simulink model "Full_System"  (R2024a)
settings: Solver=FixedStepDiscrete  StartTime=0.0  StopTime=10.0  RelTol=1e-3
undefined symbols (not defined in the file): Ion, Lithium
libraries: spsSeriesRLCBranchLib x6, spsBuckConverterLib x2, spsCurrentMeasurementLib x2, spsBatteryLib x1, spsPWMGeneratorDCDCLib x1, spsGroundLib x1, spsPVArrayLib x1, eePwmGenerator x1, spsVoltageMeasurementLib x1, spspowerguiLib x1
settings Model: Creator=KennyBoum-biha  LastModifiedBy=k_boumbi
settings DebuggingCC: UnconnectedInputMsg=warning  UnconnectedOutputMsg=warning  UnconnectedLineMsg=warning
settings ModelReferenceCC: EnableRefExpFcnMdlSchedulingChecks=on
settings RTWCC: GPUComputeCapability=3.5  DLArmComputeVersion=19.05

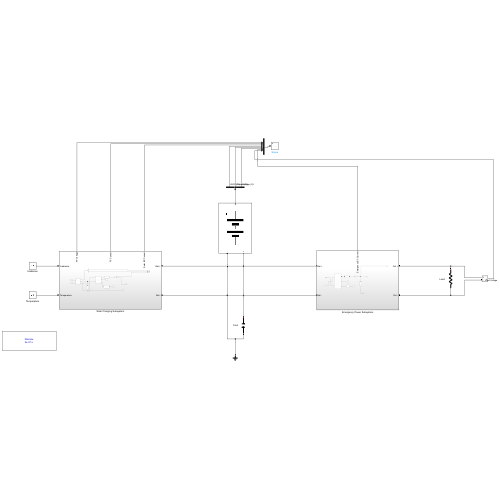
[thumbnail: Simulink's stored preview of the top-level diagram]
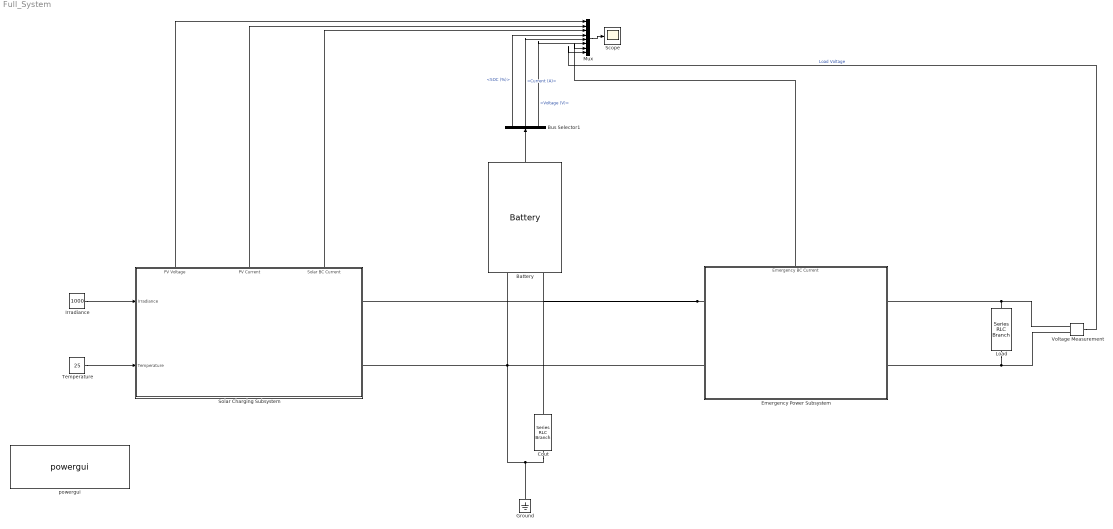
== system Full_System ==
  Battery : spsBatteryLib/Battery  BatType=Lithium-Ion  ShowTempParam=off  ThermalPreset=no  ShowAgeParam=off  NomV=48  NomQ=0.5  SOC=50  Batt_Tr=5  PresetModel=on  MaxQ=0.5  MinV=36  FullV=55.8714  Dis_rate=0.21739  R=0.96  Normal_OP=0.45217  expZone="[51.8585    0.0245652]"  current=[6.5 13 32.5]  Units=Time  Tci=20  NomT=20  T2=-30  MaxQ2=4.8  FullV2=7.1  Normal_OP2=5.655  expZone2="[6.58           1]"  Rca=0.6  ti=2000  Dp=0  Neq0=0  Tsim=1e6  Ta1=25  Qeol=5.4*0.9  Reol=0.013333*1.2  Char_age=[2.3478, 3]  Dis_age=[2.3478, 10]  N1=1500  N2=10500  N3=1000  N4=1400  Ta2=45  N5=950
  Bus Selector1 : BusSelector  OutputSignals=SOC (%),Current (A),Voltage (V)
  Cout : spsSeriesRLCBranchLib/Series RLC Branch  LConnTagsString=__new0  RConnTagsString=__new0  BranchType=C  Resistance=1  Inductance=47e-6  SetiL0=off  InitialCurrent=0  Capacitance=100e-6  Setx0=off  InitialVoltage=0  Measurements=None
  Emergency Power Subsystem : Subsystem
      settings: PortSchema="{\"entries\":[{\"content\":{\"sides\":[{\"content\":{\"connectorIds\":[\"LConn1\",\"LConn2\"]},\"type\":\"ConnectorPlacement.EquallySpacedRectSide\",\"uuid\":\"cf3750f3-3e81-4659-820f-f75c62c5389c\"},{\"content\":{\"connectorIds\":[\"RConn1\",\"RConn2\"],\"side\":\"RIGHT\"},\"type\":\"ConnectorPlacement.EquallySpacedRectSide\",\"uuid\":\"3e630a51-3c98-4ea6-b09a-757b6c47ec4c\"},{\"content\":{\"connectorIds\":[\"Out1\"],\"side\":\"TOP\"},\"type\":\"ConnectorPlacement.EquallySpacedRectSide\",\"uuid\":\"d6b0d433-2319-4baf-b8a3-4fb876102fd6\"}]},\"type\":\"ConnectorPlacement.EquallySpacedConnector\",\"uuid\":\"13c5517f-e21d-46a3-ac40-d14bb8a08b57\"}],\"packageUris\":[\"http://schema.mathworks.com/mf0/Connector/R2020b\"],\"version\":\"1.0\"}"
  Ground : spsGroundLib/Ground  LConnTagsString=a
  Irradiance : Constant  Value=1000
  Load : spsSeriesRLCBranchLib/Series RLC Branch  LConnTagsString=__new0  RConnTagsString=__new0  BranchType=R  Resistance=1.44  Inductance=1e-3  SetiL0=off  InitialCurrent=0  Capacitance=1e-6  Setx0=off  InitialVoltage=0  Measurements=None
  Mux : Mux  Inputs=8
  Scope : Scope
  Solar Charging Subsystem : Subsystem
      settings: PortSchema="{\"entries\":[{\"content\":{\"sides\":[{\"content\":{\"connectorIds\":[\"In1\",\"In2\"]},\"type\":\"ConnectorPlacement.EquallySpacedRectSide\",\"uuid\":\"cb229151-0742-4502-9ccd-990ff05f6a8c\"},{\"content\":{\"connectorIds\":[\"RConn1\",\"RConn2\"],\"side\":\"RIGHT\"},\"type\":\"ConnectorPlacement.EquallySpacedRectSide\",\"uuid\":\"9e14cc4e-58f0-4588-8f9d-a6a650a5df1b\"},{\"content\":{\"connectorIds\":[\"Out1\",\"Out2\",\"Out3\"],\"side\":\"TOP\"},\"type\":\"ConnectorPlacement.EquallySpacedRectSide\",\"uuid\":\"ec81657c-9ee6-4126-bdd0-5a56d1ba93e0\"}]},\"type\":\"ConnectorPlacement.EquallySpacedConnector\",\"uuid\":\"153089d4-0393-4364-aaa8-7b9cfec9044a\"}],\"packageUris\":[\"http://schema.mathworks.com/mf0/Connector/R2020b\"],\"version\":\"1.0\"}"
  Temperature : Constant  Value=25
  Voltage Measurement : spsVoltageMeasurementLib/Voltage Measurement  PhasorSimulation=off  OutputType=Complex  PSBequivalent=0
  powergui : spspowerguiLib/powergui  Priority=1  SimulationMode=Discrete  SampleTime=2e-7  frequency=60  Iterations=50  frequencyindice=0  Pbase=100e6  ErrMax=1e-4  UnitsV=kV  UnitsW=MW  buscounter=0  FunctionMessages=off  echomessages=off  EnableUseOfTLC=off  CurrentSourceSwitches=off  DisableSnubberDevices=off  DisableRonSwitches=off  DisableVfSwitches=off  DisplayEquations=off  AutomaticDiscreteSolvers=off  SolverType=Tustin/Backward Euler (TBE)  Interpol=off  ExternalGateDelay=off  methode=off  Ts=100  x0status=blocks  SPID=on  SwTol=0  HookPort=off  NonlinearTolerance=1e-4  nMaxIteration=100  ContinueOnMaxIteration=off  RestoreLinks=warning  ResistiveCurrentMeasurement=off  Frange=[0:2:500]  Ylog=off  Xlog=on  ShowGrid=off  save=off  variable=ZData  structure=0  ZoomFFT=off  StartTime=0.0  cycles=1  DisplayStyle=1  fundamental=60  FreqAxis=off  MaxFrequency=1000  frequencyindicesteady=1  RmsSteady=1  display=off
  wires:
  Mux/1 -> Scope/1
  Bus Selector1/1 -> Mux/4  "<SOC (%)>"
  Bus Selector1/2 -> Mux/5  "<Current (A)>"
  Bus Selector1/3 -> Mux/6  "<Voltage (V)>"
  Voltage Measurement/1 -> Mux/8  "Load Voltage"
  Irradiance/1 -> Solar Charging Subsystem/1(Irradiance)
  Temperature/1 -> Solar Charging Subsystem/2(Temperature)
  Solar Charging Subsystem/1(PV Voltage) -> Mux/1
  Solar Charging Subsystem/2(PV Current) -> Mux/2
  Solar Charging Subsystem/3(Solar BC Current) -> Mux/3
  Emergency Power Subsystem/1(Emergency BC Current) -> Mux/7
  Battery/1 -> Bus Selector1/1
  connections:
  Ground/LConn1 -- Cout/RConn1 -- Battery/LConn2 -- Emergency Power Subsystem/LConn2 -- Solar Charging Subsystem/RConn2
  Emergency Power Subsystem/LConn1 -- Cout/LConn1 -- Solar Charging Subsystem/RConn1 -- Battery/LConn1
  Load/LConn1 -- Voltage Measurement/LConn1 -- Emergency Power Subsystem/RConn1
  Load/RConn1 -- Voltage Measurement/LConn2 -- Emergency Power Subsystem/RConn2

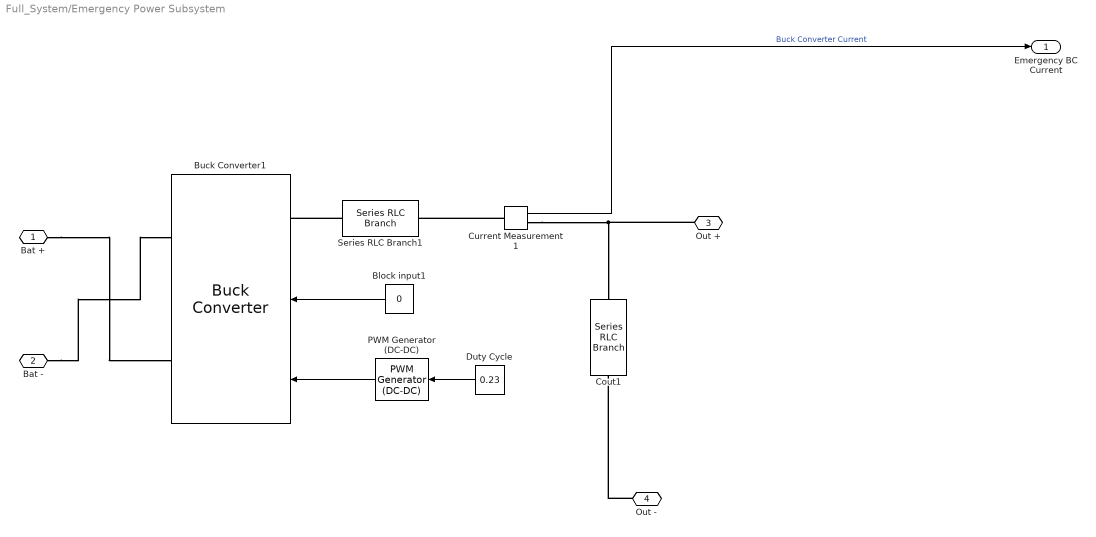
== system Full_System/Emergency Power Subsystem ==
  Block input1 : Constant  Value=0
  Buck Converter1 : spsBuckConverterLib/Buck Converter  ModelType=Switching devices  Ron=1e-3  Rs=1e6  Cs=inf  Vforward=[0,0]  Ron_Diode=1e-3  Rs_Diode=1e6  Cs_Diode=inf  Vf_Diode=1e-3  Rs_CurrentSource=inf  Ron_ACsource=1e-3
  Cout1 : spsSeriesRLCBranchLib/Series RLC Branch  LConnTagsString=__new0  RConnTagsString=__new0  BranchType=C  Resistance=1  Inductance=1e-3  SetiL0=off  InitialCurrent=0  Capacitance=220e-6  Setx0=off  InitialVoltage=0  Measurements=None
  Current Measurement1 : spsCurrentMeasurementLib/Current Measurement  PhasorSimulation=off  OutputType=Complex  PSBequivalent=0
  Duty Cycle : Constant  Value=0.23
  PWM Generator (DC-DC) : spsPWMGeneratorDCDCLib/PWM Generator (DC-DC)  Fsw=50e3  Ts=2e-7
  Series RLC Branch1 : spsSeriesRLCBranchLib/Series RLC Branch  LConnTagsString=__new0  RConnTagsString=__new0  BranchType=L  Resistance=1  Inductance=60e-6  SetiL0=off  InitialCurrent=0  Capacitance=1e-6  Setx0=off  InitialVoltage=0  Measurements=None
  Bat + : PMIOPort  Side=Left
  Bat - : PMIOPort  Port=2  Side=Left
  Out + : PMIOPort  Port=3  Side=Right
  Out - : PMIOPort  Port=4  Side=Right
  Emergency BC Current : Outport
  wires:
  Block input1/1 -> Buck Converter1/2
  Duty Cycle/1 -> PWM Generator (DC-DC)/1
  PWM Generator (DC-DC)/1 -> Buck Converter1/1
  Current Measurement1/1 -> Emergency BC Current/1  "Buck Converter Current"
  connections:
  Current Measurement1/LConn1 -- Series RLC Branch1/RConn1
  Current Measurement1/RConn1 -- Out +/RConn1 -- Cout1/LConn1
  Bat +/RConn1 -- Buck Converter1/RConn1
  Series RLC Branch1/LConn1 -- Buck Converter1/LConn1
  Bat -/RConn1 -- Buck Converter1/RConn2
  Out -/RConn1 -- Cout1/RConn1

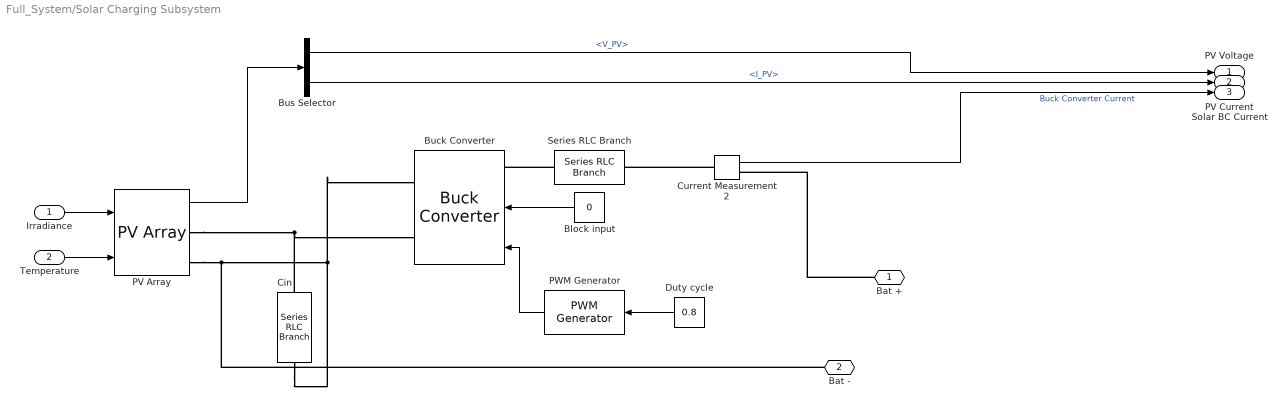
== system Full_System/Solar Charging Subsystem ==
  Irradiance : Inport
  Temperature : Inport  Port=2
  Block input : Constant  Value=0
  Buck Converter : spsBuckConverterLib/Buck Converter  ModelType=Switching devices  Ron=1e-3  Rs=1e6  Cs=inf  Vforward=[0,0]  Ron_Diode=1e-3  Rs_Diode=1e6  Cs_Diode=inf  Vf_Diode=1e-3  Rs_CurrentSource=inf  Ron_ACsource=1e-3
  Bus Selector : BusSelector  OutputSignals=V_PV,I_PV
  Cin : spsSeriesRLCBranchLib/Series RLC Branch  LConnTagsString=__new0  RConnTagsString=__new0  BranchType=C  Resistance=1  Inductance=47e-6  SetiL0=off  InitialCurrent=0  Capacitance=100e-6  Setx0=off  InitialVoltage=0  Measurements=None
  Current Measurement2 : spsCurrentMeasurementLib/Current Measurement  PhasorSimulation=off  OutputType=Complex  PSBequivalent=0
  Duty cycle : Constant  Value=0.8
  PV Array : spsPVArrayLib/PV Array  Npar=1  Nser=2  PlotType=array @ 1000 W/m2 & specified temperatures  S_vec="[ 1000  500  100 ]"  Temp_C_vec="[ 45 25  ]"  ModuleName=User-defined  PlotWhenSelected=off  Pm=213.15  Ncell=60  Voc=36.3  Isc=7.84  Vm=29  Im=7.35  beta_Voc_pc=-0.36099  alpha_Isc_pc=0.102  beta_Voc=-0.13104  alpha_Isc=0.0079968  IL=7.8654  I0=2.9273e-10  nI=0.98119  Rsh=313.0553  Rs=0.39381  RobustModel=off  RobustCellTemperature=313.3991  BAL=on  Tc=1e-6  Tfilter=5e-5
  PWM Generator : eePwmGenerator/PWM Generator  CarrCount=Up  Tper=0.001  Tdelay=0  Ts=2e-7
  Series RLC Branch : spsSeriesRLCBranchLib/Series RLC Branch  LConnTagsString=__new0  RConnTagsString=__new0  BranchType=L  Resistance=1  Inductance=47e-6  SetiL0=off  InitialCurrent=0  Capacitance=1e-6  Setx0=off  InitialVoltage=0  Measurements=None
  Bat + : PMIOPort  Side=Right
  Bat - : PMIOPort  Port=2  Side=Right
  PV Voltage : Outport
  PV Current : Outport  Port=2
  Solar BC Current : Outport  Port=3
  wires:
  Duty cycle/1 -> PWM Generator/1
  Block input/1 -> Buck Converter/2
  PWM Generator/1 -> Buck Converter/1
  PV Array/1 -> Bus Selector/1
  Temperature/1 -> PV Array/2
  Bus Selector/2 -> PV Current/1  "<I_PV>"
  Bus Selector/1 -> PV Voltage/1  "<V_PV>"
  Irradiance/1 -> PV Array/1
  Current Measurement2/1 -> Solar BC Current/1  "Buck Converter Current"
  connections:
  PV Array/RConn2 -- Bat -/RConn1 -- Cin/RConn1 -- Buck Converter/RConn2
  Current Measurement2/LConn1 -- Series RLC Branch/RConn1
  PV Array/RConn1 -- Cin/LConn1 -- Buck Converter/RConn1
  Series RLC Branch/LConn1 -- Buck Converter/LConn1
  Bat +/RConn1 -- Current Measurement2/RConn1
